simulink model "reinforcemen_model_realtest"  (R2023b)
settings: Solver=FixedStepAuto  StartTime=0.0  StopTime=inf  FixedStep=0.05  RelTol=1e-3
undefined symbols (not defined in the file or in its folder): saved_agent, Ts
libraries: arduinolib x10, rllib x5, dspstat3 x5, dxlSimLibrary x4, simulink x2
settings Model: SimulationMode=accelerator  ExtModeTrigDuration=2  VariantFading=off  Creator=MSI PC  LastModifiedBy=Yuk
settings OptimizationCC: EnhancedBackFolding=on  PassReuseOutputArgsAs=Individual arguments  ZeroExternalMemoryAtStartup=off  ZeroInternalMemoryAtStartup=off  MaxStackSize=64  OptimizeBlockOrder=speed  DifferentSizesBufferReuse=on  OptimizationCustomize=off  EfficientTunableParamExpr=on
settings DebuggingCC: MultiTaskRateTransMsg=warning  ParameterPrecisionLossMsg=none  ParameterTunabilityLossMsg=error  UnconnectedInputMsg=warning  UnconnectedOutputMsg=warning  UnconnectedLineMsg=warning
settings HardwareCC: ProdBitPerInt=16  ProdBitPerPointer=16  ProdBitPerSizeT=16  ProdBitPerPtrDiffT=16  ProdLargestAtomicFloat=None  ProdWordSize=8  ProdHWDeviceType=Atmel->AVR
settings ModelReferenceCC: EnableRefExpFcnMdlSchedulingChecks=on
settings SFSimCC: MATLABDynamicMemAlloc=off
settings RTWCC: Description=Embedded Coder  SystemTargetFile=ert.tlc  HardwareBoard=Arduino Uno  TemplateMakefile=ert_default_tmf  Toolchain=Arduino AVR  BuildConfiguration=Faster Runs  DLArmComputeVersion=19.05
settings CodeAppCC: ForceParamTrailComments=on  IgnoreCustomStorageClasses=off  OperatorAnnotations=on  SimulinkDataObjDesc=on  SFDataObjDesc=on  InsertBlockDesc=on
settings ERTTargetCC: SupportContinuousTime=on  SupportVariableSizeSignals=on  ExtModeTransport=3  ExtModeStaticAlloc=on  ExtModeAutomaticAllocSize=off  ExtModeStaticAllocSize=250  ExtModeMexFile=ext_xcp  ExtModeIntrfLevel=Level2 - Open

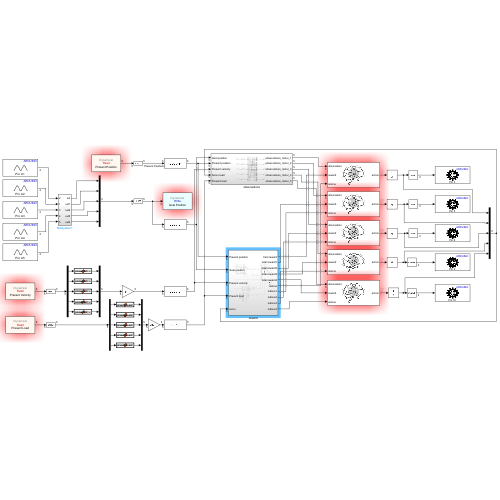
[thumbnail: Simulink's stored preview of the top-level diagram]
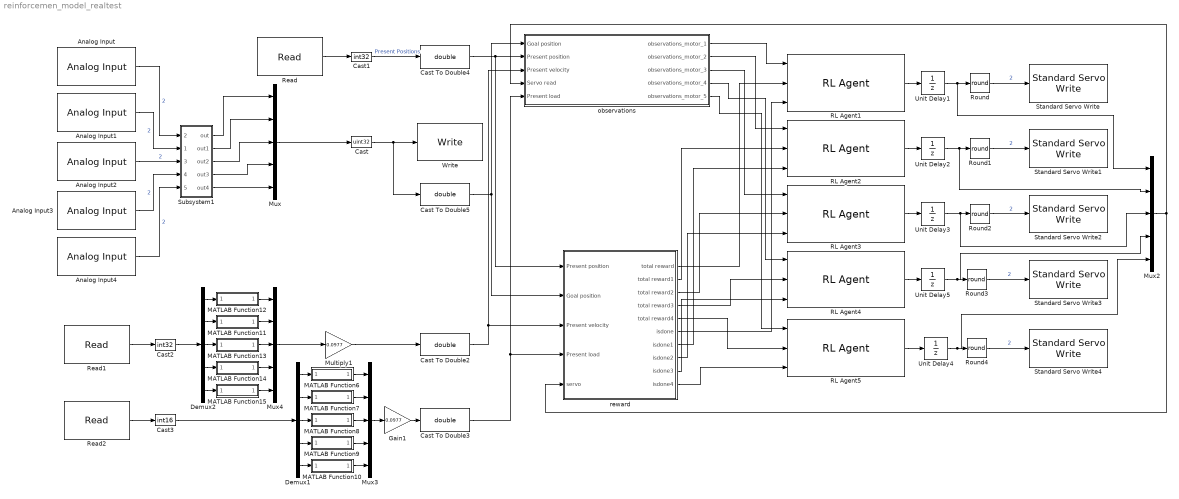
== system reinforcemen_model_realtest ==
  Analog Input : arduinolib/Analog Input  pinNumber=1  ReadResultsOnly=off  ConversionTriggerSource=Software  ExternalTriggerType=uint32( 0 )  OutputDataType=uint16  EnableConversionCompleteNotify=off  EnableOuputStatus=off  SampleTime=0.05  blockPlatform=arduino
  Analog Input1 : arduinolib/Analog Input  pinNumber=2  ReadResultsOnly=off  ConversionTriggerSource=Software  ExternalTriggerType=uint32( 0 )  OutputDataType=uint16  EnableConversionCompleteNotify=off  EnableOuputStatus=off  SampleTime=0.05  blockPlatform=arduino
  Analog Input2 : arduinolib/Analog Input  pinNumber=3  ReadResultsOnly=off  ConversionTriggerSource=Software  ExternalTriggerType=uint32( 0 )  OutputDataType=uint16  EnableConversionCompleteNotify=off  EnableOuputStatus=off  SampleTime=0.05  blockPlatform=arduino
  Analog Input3 : arduinolib/Analog Input  pinNumber=4  ReadResultsOnly=off  ConversionTriggerSource=Software  ExternalTriggerType=uint32( 0 )  OutputDataType=uint16  EnableConversionCompleteNotify=off  EnableOuputStatus=off  SampleTime=0.05  blockPlatform=arduino
  Analog Input4 : arduinolib/Analog Input  pinNumber=5  ReadResultsOnly=off  ConversionTriggerSource=Software  ExternalTriggerType=uint32( 0 )  OutputDataType=uint16  EnableConversionCompleteNotify=off  EnableOuputStatus=off  SampleTime=0.05  blockPlatform=arduino
  Cast : DataTypeConversion  OutMin=0  OutMax=2097150  OutDataTypeStr=uint32  SaturateOnIntegerOverflow=off  RndMeth=Floor
  Cast To Double{2..5} (4 alike) : DataTypeConversion  OutDataTypeStr=double  SaturateOnIntegerOverflow=off  RndMeth=Floor
  Cast1 : DataTypeConversion  OutDataTypeStr=int32  SaturateOnIntegerOverflow=off  RndMeth=Floor
  Cast2 : DataTypeConversion  OutDataTypeStr=int32  SaturateOnIntegerOverflow=off  RndMeth=Floor
  Cast3 : DataTypeConversion  OutDataTypeStr=int16  SaturateOnIntegerOverflow=off  RndMeth=Floor
  Demux1 : Demux  Outputs=5
  Demux2 : Demux  Outputs=5
  Gain1 : Gain  Gain=0.0977
  MATLAB Function10 : MATLAB Function  TreatAsAtomicUnit=on
  MATLAB Function11 : MATLAB Function  TreatAsAtomicUnit=on
  MATLAB Function12 : MATLAB Function  TreatAsAtomicUnit=on
  MATLAB Function13 : MATLAB Function  TreatAsAtomicUnit=on
  MATLAB Function14 : MATLAB Function  TreatAsAtomicUnit=on
  MATLAB Function15 : MATLAB Function  TreatAsAtomicUnit=on
  MATLAB Function6 : MATLAB Function  TreatAsAtomicUnit=on
  MATLAB Function7 : MATLAB Function  TreatAsAtomicUnit=on
  MATLAB Function8 : MATLAB Function  TreatAsAtomicUnit=on
  MATLAB Function9 : MATLAB Function  TreatAsAtomicUnit=on
  Multiply1 : Gain  Gain=0.0977  OutDataTypeStr=double
  Mux{,2..4} (4 alike) : Mux  Inputs=5
  RL Agent1 : rllib/RL Agent  Agent=saved_agent(1,1)  ExternalActionAsInput=off  ProvideLastAction=off  ProvideCumRwd=off  TreatAsDirectFeedthrough=on  UseStrictObservationDataTypes=off
  RL Agent2 : rllib/RL Agent  Agent=saved_agent(1,2)  ExternalActionAsInput=off  ProvideLastAction=off  ProvideCumRwd=off  TreatAsDirectFeedthrough=on  UseStrictObservationDataTypes=off
  RL Agent3 : rllib/RL Agent  Agent=saved_agent(1,3)  ExternalActionAsInput=off  ProvideLastAction=off  ProvideCumRwd=off  TreatAsDirectFeedthrough=on  UseStrictObservationDataTypes=off
  RL Agent4 : rllib/RL Agent  Agent=saved_agent(1,4)  ExternalActionAsInput=off  ProvideLastAction=off  ProvideCumRwd=off  TreatAsDirectFeedthrough=on  UseStrictObservationDataTypes=off
  RL Agent5 : rllib/RL Agent  Agent=saved_agent(1,5)  ExternalActionAsInput=off  ProvideLastAction=off  ProvideCumRwd=off  TreatAsDirectFeedthrough=on  UseStrictObservationDataTypes=off
  Read : dxlSimLibrary/Read  lib_name=lib_name  port_num=port_num  protocol_version=protocol_version  ids=motor_IDs  models=motor_models  select=Present Position  Ts=Ts
  Read1 : dxlSimLibrary/Read  lib_name=lib_name  port_num=port_num  protocol_version=protocol_version  ids=motor_IDs  models=motor_models  select=Present Velocity  Ts=Ts
  Read2 : dxlSimLibrary/Read  lib_name=lib_name  port_num=port_num  protocol_version=protocol_version  ids=motor_IDs  models=motor_models  select=Present Load  Ts=Ts
  Round{,1..4} (5 alike) : Rounding  Operator=round
  Standard Servo Write : arduinolib/Standard Servo Write  pinNumber=3  ServoIndex=0  blockPlatform=ARDUINO
  Standard Servo Write1 : arduinolib/Standard Servo Write  pinNumber=5  ServoIndex=1  blockPlatform=ARDUINO
  Standard Servo Write2 : arduinolib/Standard Servo Write  pinNumber=6  ServoIndex=2  blockPlatform=ARDUINO
  Standard Servo Write3 : arduinolib/Standard Servo Write  pinNumber=9  ServoIndex=3  blockPlatform=ARDUINO
  Standard Servo Write4 : arduinolib/Standard Servo Write  pinNumber=10  ServoIndex=4  blockPlatform=ARDUINO
  Subsystem1 : Subsystem
  Unit Delay1 : UnitDelay  SampleTime=-1  HasFrameUpgradeWarning=on
  Unit Delay{2..5} (4 alike) : UnitDelay  InitialCondition=180  SampleTime=-1  HasFrameUpgradeWarning=on
  Write : dxlSimLibrary/Write  lib_name=lib_name  port_num=port_num  protocol_version=protocol_version  ids=motor_IDs  models=motor_models  select=Goal Position  Ts=Ts
  observations : Subsystem
  reward : Subsystem
  wires:
  observations/5(observations_motor_5) -> RL Agent5/1
  Cast2/1 -> Demux2/1
  Cast3/1 -> Demux1/1
  Read1/1 -> Cast2/1
  Read2/1 -> Cast3/1
  Analog Input/1 -> Subsystem1/1(2)  "2"
  Analog Input1/1 -> Subsystem1/2(1)  "2"
  Analog Input4/1 -> Subsystem1/5(5)  "2"
  Analog Input2/1 -> Subsystem1/3(3)  "2"
  Analog Input3/1 -> Subsystem1/4(4)  "2"
  Demux2/1 -> MATLAB Function12/1(presentVel)
  Demux2/5 -> MATLAB Function15/1(presentVel)
  Demux2/4 -> MATLAB Function14/1(presentVel)
  Demux2/3 -> MATLAB Function13/1(presentVel)
  Demux2/2 -> MATLAB Function11/1(presentVel)
  Demux1/3 -> MATLAB Function8/1(presentLoad)
  Demux1/2 -> MATLAB Function7/1(presentLoad)
  Demux1/1 -> MATLAB Function6/1(presentLoad)
  Gain1/1 -> Cast To Double3/1
  Demux1/5 -> MATLAB Function10/1(presentLoad)
  Demux1/4 -> MATLAB Function9/1(presentLoad)
  Mux/1 -> Cast/1
  Subsystem1/5(out4) -> Mux/5
  Subsystem1/1(out) -> Mux/1
  Subsystem1/3(out2) -> Mux/3
  Subsystem1/2(out1) -> Mux/2
  Subsystem1/4(out3) -> Mux/4
  MATLAB Function14/1(convertedVel) -> Mux4/4
  MATLAB Function13/1(convertedVel) -> Mux4/3
  MATLAB Function11/1(convertedVel) -> Mux4/2
  MATLAB Function12/1(convertedVel) -> Mux4/1
  reward/6(isdone) -> RL Agent1/3
  Multiply1/1 -> Cast To Double2/1
  MATLAB Function15/1(convertedVel) -> Mux4/5
  MATLAB Function10/1(convertedLoad) -> Mux3/5
  MATLAB Function8/1(convertedLoad) -> Mux3/3
  MATLAB Function7/1(convertedLoad) -> Mux3/2
  MATLAB Function6/1(convertedLoad) -> Mux3/1
  RL Agent2/1 -> Unit Delay2/1
  MATLAB Function9/1(convertedLoad) -> Mux3/4
  Read/1 -> Cast1/1
  Mux4/1 -> Multiply1/1
  Mux3/1 -> Gain1/1
  reward/3(total reward2) -> RL Agent3/2
  Cast1/1 -> Cast To Double4/1  "Present Positions"
  reward/4(total reward3) -> RL Agent4/2
  Cast/1 -> Write/1, Cast To Double5/1
  Cast To Double5/1 -> reward/2(Goal position), observations/1(Goal position)
  reward/5(total reward4) -> RL Agent5/2
  Cast To Double4/1 -> reward/1(Present position), observations/2(Present position)
  Cast To Double2/1 -> reward/3(Present velocity), observations/3(Present velocity)
  RL Agent3/1 -> Unit Delay3/1
  observations/1(observations_motor_1) -> RL Agent1/1
  observations/2(observations_motor_2) -> RL Agent2/1
  observations/3(observations_motor_3) -> RL Agent3/1
  observations/4(observations_motor_4) -> RL Agent4/1
  reward/1(total reward) -> RL Agent1/2
  reward/2(total reward1) -> RL Agent2/2
  reward/7(isdone1) -> RL Agent2/3
  reward/8(isdone2) -> RL Agent3/3
  reward/9(isdone3) -> RL Agent4/3
  reward/10(isdone4) -> RL Agent5/3
  RL Agent4/1 -> Unit Delay5/1
  RL Agent5/1 -> Unit Delay4/1
  Round1/1 -> Standard Servo Write1/1  "2"
  RL Agent1/1 -> Unit Delay1/1
  Round2/1 -> Standard Servo Write2/1  "2"
  Round3/1 -> Standard Servo Write3/1  "2"
  Round4/1 -> Standard Servo Write4/1  "2"
  Round/1 -> Standard Servo Write/1  "2"
  Mux2/1 -> reward/5(servo), observations/4(Servo read)
  Unit Delay5/1 -> Mux2/4, Round3/1
  Unit Delay4/1 -> Mux2/5, Round4/1
  Unit Delay1/1 -> Round/1, Mux2/1
  Cast To Double3/1 -> reward/4(Present load), observations/5(Present load)
  Unit Delay3/1 -> Mux2/3, Round2/1
  Unit Delay2/1 -> Mux2/2, Round1/1

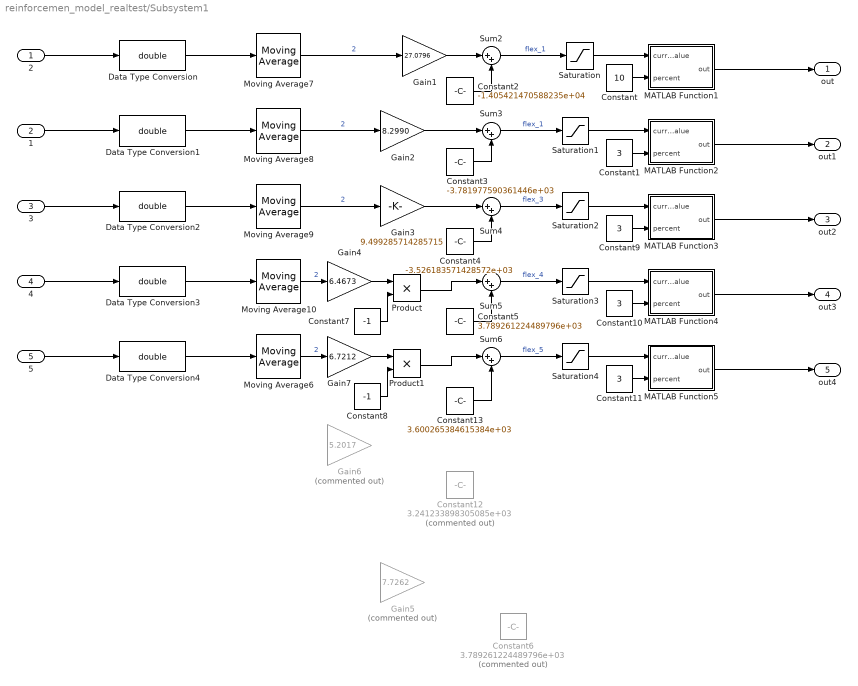
== system reinforcemen_model_realtest/Subsystem1 ==
  2 : Inport
  1 : Inport  Port=2
  3 : Inport  Port=3
  4 : Inport  Port=4
  5 : Inport  Port=5
  Constant : Constant  Value=10
  Constant{1,9..11} (4 alike) : Constant  Value=3
  Constant12 : Constant  Commented=on  Value=3.241233898305085e+03
  Constant13 : Constant  Value=3.600265384615384e+03
  Constant2 : Constant  Value=-1.405421470588235e+04
  Constant3 : Constant  Value=-3.781977590361446e+03
  Constant4 : Constant  Value=-3.526183571428572e+03
  Constant5 : Constant  Value=3.789261224489796e+03
  Constant6 : Constant  Commented=on  Value=3.789261224489796e+03
  Constant7 : Constant  Value=-1
  Constant8 : Constant  Value=-1
  Data Type Conversion{,1..4} (5 alike) : DataTypeConversion  OutDataTypeStr=double  SaturateOnIntegerOverflow=off  RndMeth=Floor
  Gain1 : Gain  Gain=27.0796
  Gain2 : Gain  Gain=8.2990
  Gain3 : Gain  Gain=9.499285714285715
  Gain4 : Gain  Gain=6.4673
  Gain5 : Gain  Commented=on  Gain=7.7262
  Gain6 : Gain  Commented=on  Gain=5.2017
  Gain7 : Gain  Gain=6.7212
  MATLAB Function1 : MATLAB Function  TreatAsAtomicUnit=on
  MATLAB Function2 : MATLAB Function  TreatAsAtomicUnit=on
  MATLAB Function3 : MATLAB Function  TreatAsAtomicUnit=on
  MATLAB Function4 : MATLAB Function  TreatAsAtomicUnit=on
  MATLAB Function5 : MATLAB Function  TreatAsAtomicUnit=on
  Moving Average{6..10} (5 alike) : dspstat3/Moving Average  Method=Sliding window  ForgettingFactorPort=off  SpecifyWindowLength=on  WindowLength=3  OverlapLength=2  AllowArbitraryInputLength=off  ForgettingFactor=0.9  SimulateUsing=Code generation
  Product : Product
  Product1 : Product
  Saturation : Saturate  UpperLimit=920.7  LowerLimit=0
  Saturation1 : Saturate  UpperLimit=716.1  LowerLimit=27.28
  Saturation2 : Saturate  UpperLimit=640  LowerLimit=17.05
  Saturation3 : Saturate  UpperLimit=988.9  LowerLimit=375.1
  Saturation4 : Saturate  UpperLimit=1005.9  LowerLimit=306.9
  Sum{2..6} (5 alike) : Sum  Inputs=|++
  out : Outport
  out1 : Outport  Port=2
  out2 : Outport  Port=3
  out3 : Outport  Port=4
  out4 : Outport  Port=5
  wires:
  3/1 -> Data Type Conversion2/1
  5/1 -> Data Type Conversion4/1
  MATLAB Function4/1(out) -> out3/1
  MATLAB Function1/1(out) -> out/1
  MATLAB Function2/1(out) -> out1/1
  1/1 -> Data Type Conversion1/1
  Constant5/1 -> Sum5/2
  Constant9/1 -> MATLAB Function3/2(percent)
  Constant/1 -> MATLAB Function1/2(percent)
  Constant10/1 -> MATLAB Function4/2(percent)
  Sum5/1 -> Saturation3/1  "flex_4"
  Saturation/1 -> MATLAB Function1/1(currentValue)
  4/1 -> Data Type Conversion3/1
  Constant4/1 -> Sum4/2
  Moving Average6/1 -> Gain7/1  "2"
  Gain2/1 -> Sum3/1
  Constant1/1 -> MATLAB Function2/2(percent)
  MATLAB Function5/1(out) -> out4/1
  Constant8/1 -> Product1/2
  Moving Average9/1 -> Gain3/1  "2"
  Constant3/1 -> Sum3/2
  Product1/1 -> Sum6/1
  Saturation4/1 -> MATLAB Function5/1(currentValue)
  MATLAB Function3/1(out) -> out2/1
  Moving Average7/1 -> Gain1/1  "2"
  Data Type Conversion2/1 -> Moving Average9/1
  Data Type Conversion/1 -> Moving Average7/1
  Data Type Conversion4/1 -> Moving Average6/1
  Gain1/1 -> Sum2/1
  Saturation3/1 -> MATLAB Function4/1(currentValue)
  Moving Average8/1 -> Gain2/1  "2"
  Gain4/1 -> Product/1
  Constant11/1 -> MATLAB Function5/2(percent)
  Sum4/1 -> Saturation2/1  "flex_3"
  Saturation2/1 -> MATLAB Function3/1(currentValue)
  Data Type Conversion1/1 -> Moving Average8/1
  Sum3/1 -> Saturation1/1  "flex_1"
  Sum2/1 -> Saturation/1  "flex_1"
  Saturation1/1 -> MATLAB Function2/1(currentValue)
  Constant7/1 -> Product/2
  2/1 -> Data Type Conversion/1
  Constant2/1 -> Sum2/2
  Gain3/1 -> Sum4/1
  Sum6/1 -> Saturation4/1  "flex_5"
  Gain7/1 -> Product1/1
  Data Type Conversion3/1 -> Moving Average10/1
  Moving Average10/1 -> Gain4/1  "2"
  Constant13/1 -> Sum6/2
  Product/1 -> Sum5/1

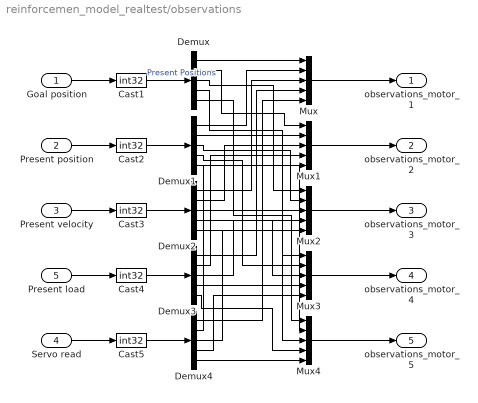
== system reinforcemen_model_realtest/observations ==
  Goal position : Inport
  Present position : Inport  Port=2
  Present velocity : Inport  Port=3
  Servo read : Inport  Port=4
  Present load : Inport  Port=5
  Cast{1..5} (5 alike) : DataTypeConversion  OutDataTypeStr=int32  SaturateOnIntegerOverflow=off  RndMeth=Floor
  Demux{,1..4} (5 alike) : Demux  Outputs=5
  Mux{,1..4} (5 alike) : Mux  Inputs=5
  observations_motor_1 : Outport
  observations_motor_2 : Outport  Port=2
  observations_motor_3 : Outport  Port=3
  observations_motor_4 : Outport  Port=4
  observations_motor_5 : Outport  Port=5
  wires:
  Goal position/1 -> Cast1/1
  Present position/1 -> Cast2/1
  Present velocity/1 -> Cast3/1
  Present load/1 -> Cast4/1
  Servo read/1 -> Cast5/1
  Demux/1 -> Mux/1
  Demux1/1 -> Mux/2
  Demux2/1 -> Mux/3
  Demux3/1 -> Mux/4
  Demux4/1 -> Mux/5
  Demux/2 -> Mux1/1
  Demux1/2 -> Mux1/2
  Demux2/2 -> Mux1/3
  Demux3/2 -> Mux1/4
  Demux4/2 -> Mux1/5
  Demux/3 -> Mux2/1
  Demux1/3 -> Mux2/2
  Demux2/3 -> Mux2/3
  Demux3/3 -> Mux2/4
  Demux4/3 -> Mux2/5
  Demux/4 -> Mux3/1
  Demux1/4 -> Mux3/2
  Demux2/4 -> Mux3/3
  Demux3/4 -> Mux3/4
  Demux4/4 -> Mux3/5
  Demux/5 -> Mux4/1
  Demux1/5 -> Mux4/2
  Demux2/5 -> Mux4/3
  Demux3/5 -> Mux4/4
  Demux4/5 -> Mux4/5
  Mux/1 -> observations_motor_1/1
  Mux1/1 -> observations_motor_2/1
  Mux2/1 -> observations_motor_3/1
  Mux3/1 -> observations_motor_4/1
  Mux4/1 -> observations_motor_5/1
  Cast2/1 -> Demux1/1
  Cast3/1 -> Demux2/1
  Cast4/1 -> Demux3/1
  Cast5/1 -> Demux4/1
  Cast1/1 -> Demux/1  "Present Positions"

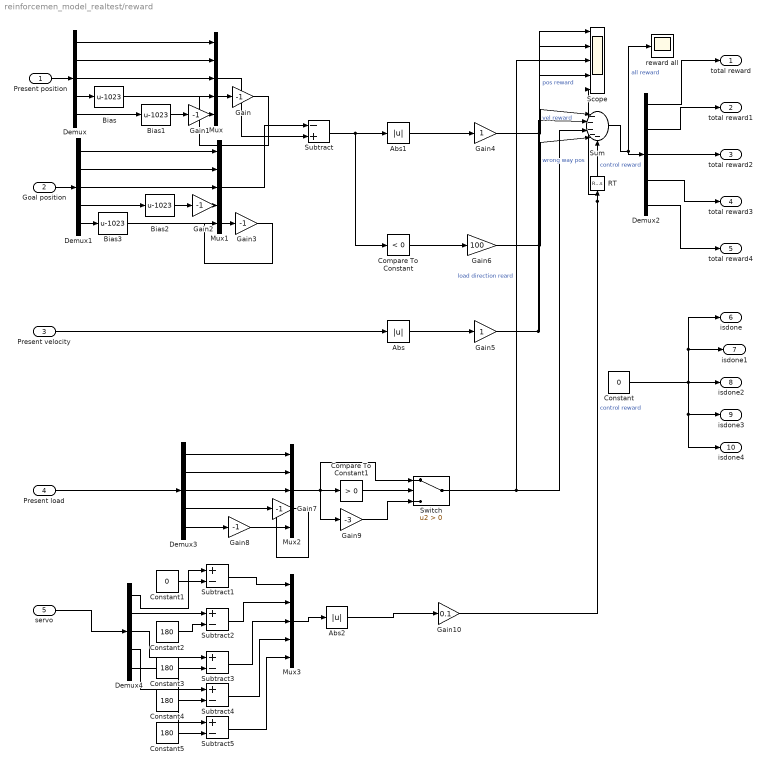
== system reinforcemen_model_realtest/reward ==
  Present position : Inport
  Goal position : Inport  Port=2
  Present velocity : Inport  Port=3
  Present load : Inport  Port=4
  servo : Inport  Port=5
  Abs : Abs  SaturateOnIntegerOverflow=off
  Abs1 : Abs  SaturateOnIntegerOverflow=off
  Abs2 : Abs  SaturateOnIntegerOverflow=off
  Bias{,1..3} (4 alike) : Bias  Bias=-1023  SaturateOnIntegerOverflow=off
  Compare To Constant : simulink/Logic and Bit Operations/Compare To Constant  relop=<  const=0  OutDataTypeStr=boolean
  Compare To Constant1 : simulink/Logic and Bit Operations/Compare To Constant  relop=>  const=0  OutDataTypeStr=boolean
  Constant : Constant  Value=0
  Constant1 : Constant  Value=0
  Constant{2..5} (4 alike) : Constant  Value=180
  Demux{,1..4} (5 alike) : Demux  Outputs=5
  Gain{,1..3,7..8} (6 alike) : Gain  Gain=-1
  Gain10 : Gain  Gain=0.1
  Gain4 : Gain
  Gain5 : Gain
  Gain6 : Gain  Gain=100
  Gain9 : Gain  Gain=-3
  Mux{,1..3} (4 alike) : Mux  Inputs=5
  RT : RateTransition  OutPortSampleTime=0.05
  Scope : Scope  NumInputPorts=5
  Subtract : Sum  Inputs=-+
  Subtract{1..5} (5 alike) : Sum  Inputs=+-
  Sum : Sum  Inputs=|-----
  Switch : Switch  Criteria=u2 > Threshold  SaturateOnIntegerOverflow=off  InputSameDT=off
  reward all : Scope
  total reward : Outport
  total reward1 : Outport  Port=2
  total reward2 : Outport  Port=3
  total reward3 : Outport  Port=4
  total reward4 : Outport  Port=5
  isdone : Outport  Port=6
  isdone1 : Outport  Port=7
  isdone2 : Outport  Port=8
  isdone3 : Outport  Port=9
  isdone4 : Outport  Port=10
  wires:
  Present velocity/1 -> Abs/1
  Present position/1 -> Demux/1
  Demux/5 -> Bias1/1
  Demux/4 -> Bias/1
  Demux/3 -> Mux/3
  Demux/2 -> Mux/2
  Demux/1 -> Mux/1
  Bias/1 -> Gain/1
  Bias1/1 -> Gain1/1
  Gain/1 -> Mux/4
  Gain1/1 -> Mux/5
  Gain3/1 -> Mux1/5
  Gain2/1 -> Mux1/4
  Bias3/1 -> Gain3/1
  Bias2/1 -> Gain2/1
  Demux1/1 -> Mux1/1
  Demux1/2 -> Mux1/2
  Demux1/3 -> Mux1/3
  Demux1/4 -> Bias2/1
  Demux1/5 -> Bias3/1
  Goal position/1 -> Demux1/1
  Mux1/1 -> Subtract/1
  Mux/1 -> Subtract/2
  Subtract/1 -> Compare To Constant/1, Abs1/1
  Abs1/1 -> Gain4/1
  Gain4/1 -> Scope/1, Sum/1  "pos reward"
  Abs/1 -> Gain5/1
  Gain5/1 -> Scope/2, Sum/2  "vel reward"
  Present load/1 -> Demux3/1
  Compare To Constant/1 -> Gain6/1
  Gain6/1 -> Scope/4, Sum/4  "wrong way pos"
  Constant/1 -> isdone4/1, isdone3/1, isdone/1, isdone1/1, isdone2/1
  Sum/1 -> Demux2/1, reward all/1  "all reward"
  Demux2/3 -> total reward2/1
  Demux2/2 -> total reward1/1
  Demux2/1 -> total reward/1
  Demux2/4 -> total reward3/1
  Demux2/5 -> total reward4/1
  Demux3/4 -> Gain7/1
  Demux3/1 -> Mux2/1
  Demux3/3 -> Mux2/3
  Demux3/5 -> Gain8/1
  Gain7/1 -> Mux2/4
  Demux3/2 -> Mux2/2
  Gain8/1 -> Mux2/5
  Mux2/1 -> Gain9/1, Switch/1, Compare To Constant1/1
  Compare To Constant1/1 -> Switch/2
  Gain9/1 -> Switch/3
  Switch/1 -> Scope/3, Sum/3  "load direction reard"
  servo/1 -> Demux4/1
  Abs2/1 -> Gain10/1
  Demux4/5 -> Subtract5/1
  Demux4/2 -> Subtract2/1
  Demux4/4 -> Subtract4/1
  Demux4/1 -> Subtract1/1
  Demux4/3 -> Subtract3/1
  Constant1/1 -> Subtract1/2
  Constant2/1 -> Subtract2/2
  Constant3/1 -> Subtract3/2
  Constant4/1 -> Subtract4/2
  Constant5/1 -> Subtract5/2
  Subtract3/1 -> Mux3/3
  Subtract2/1 -> Mux3/2
  Subtract1/1 -> Mux3/1
  Subtract4/1 -> Mux3/4
  Subtract5/1 -> Mux3/5
  Mux3/1 -> Abs2/1
  Gain10/1 -> Scope/5, RT/1  "control reward"
  RT/1 -> Sum/5  "control reward"

== matlab function reinforcemen_model_realtest/MATLAB Function14 ==
  data: presentVel input; convertedVel output
function convertedVel = convertVel(presentVel)
% Convert Dynamixel present load data from 0-2047 to -1023 to 1023
% 0-1023 remains as is, 1024-2047 is mapped to 0 to -1023

if presentVel >= 1024
    convertedVel = -(presentVel - 1024);
else
    convertedVel = presentVel;
end
end

== matlab function reinforcemen_model_realtest/MATLAB Function15 ==
  data: presentVel input; convertedVel output
function convertedVel = convertVel(presentVel)
% Convert Dynamixel present load data from 0-2047 to -1023 to 1023
% 0-1023 remains as is, 1024-2047 is mapped to 0 to -1023

if presentVel >= 1024
    convertedVel = -(presentVel - 1024);
else
    convertedVel = presentVel;
end
end

== matlab function reinforcemen_model_realtest/Subsystem1/MATLAB Function1 ==
  data: currentValue input; out output; percent input
function out = customDeadZone(currentValue,percent)
    % 지속적인 상태 유지를 위한 영구 변수 선언
    persistent lastValue
    if isempty(lastValue)
        lastValue = currentValue; % 최초 실행 시 초기값 설정
    end
    
    % 변화 임계값 설정
    threshold = (percent*682)/100;
    
    % 현재 값과 이전 값의 차이가 임계값보다 크면 업데이트
    if abs(currentValue - lastValue) > threshold
        lastValue = currentValue; % 값 업데이트
    end
    
    % 출력
    out = lastValue;
end

== matlab function reinforcemen_model_realtest/Subsystem1/MATLAB Function3 ==
  data: currentValue input; out output; percent input
function out = customDeadZone(currentValue,percent)
    % 지속적인 상태 유지를 위한 영구 변수 선언
    persistent lastValue
    if isempty(lastValue)
        lastValue = currentValue; % 최초 실행 시 초기값 설정
    end
    
    % 변화 임계값 설정
    threshold = (percent*682)/100;
    
    % 현재 값과 이전 값의 차이가 임계값보다 크면 업데이트
    if abs(currentValue - lastValue) > threshold
        lastValue = currentValue; % 값 업데이트
    end
    
    % 출력
    out = lastValue;
end

== matlab function reinforcemen_model_realtest/Subsystem1/MATLAB Function4 ==
  data: currentValue input; out output; percent input
function out = customDeadZone(currentValue,percent)
    % 지속적인 상태 유지를 위한 영구 변수 선언
    persistent lastValue
    if isempty(lastValue)
        lastValue = currentValue; % 최초 실행 시 초기값 설정
    end
    
    % 변화 임계값 설정
    threshold = (percent*682)/100;
    
    % 현재 값과 이전 값의 차이가 임계값보다 크면 업데이트
    if abs(currentValue - lastValue) > threshold
        lastValue = currentValue; % 값 업데이트
    end
    
    % 출력
    out = lastValue;
end

== matlab function reinforcemen_model_realtest/Subsystem1/MATLAB Function5 ==
  data: currentValue input; out output; percent input
function out = customDeadZone(currentValue,percent)
    % 지속적인 상태 유지를 위한 영구 변수 선언
    persistent lastValue
    if isempty(lastValue)
        lastValue = currentValue; % 최초 실행 시 초기값 설정
    end
    
    % 변화 임계값 설정
    threshold = (percent*682)/100;
    
    % 현재 값과 이전 값의 차이가 임계값보다 크면 업데이트
    if abs(currentValue - lastValue) > threshold
        lastValue = currentValue; % 값 업데이트
    end
    
    % 출력
    out = lastValue;
end

== matlab function reinforcemen_model_realtest/MATLAB Function6 ==
  data: presentLoad input; convertedLoad output
function convertedLoad = convertLoad(presentLoad)
% Convert Dynamixel present load data from 0-2047 to -1023 to 1023
% 0-1023 remains as is, 1024-2047 is mapped to 0 to -1023

if presentLoad >= 1024
    convertedLoad = -(presentLoad - 1024);
else
    convertedLoad = presentLoad;
end
end

== matlab function reinforcemen_model_realtest/MATLAB Function7 ==
  data: presentLoad input; convertedLoad output
function convertedLoad = convertLoad(presentLoad)
% Convert Dynamixel present load data from 0-2047 to -1023 to 1023
% 0-1023 remains as is, 1024-2047 is mapped to 0 to -1023

if presentLoad >= 1024
    convertedLoad = -(presentLoad - 1024);
else
    convertedLoad = presentLoad;
end
end

== matlab function reinforcemen_model_realtest/MATLAB Function8 ==
  data: presentLoad input; convertedLoad output
function convertedLoad = convertLoad(presentLoad)
% Convert Dynamixel present load data from 0-2047 to -1023 to 1023
% 0-1023 remains as is, 1024-2047 is mapped to 0 to -1023

if presentLoad >= 1024
    convertedLoad = -(presentLoad - 1024);
else
    convertedLoad = presentLoad;
end
end

== matlab function reinforcemen_model_realtest/MATLAB Function9 ==
  data: presentLoad input; convertedLoad output
function convertedLoad = convertLoad(presentLoad)
% Convert Dynamixel present load data from 0-2047 to -1023 to 1023
% 0-1023 remains as is, 1024-2047 is mapped to 0 to -1023

if presentLoad >= 1024
    convertedLoad = -(presentLoad - 1024);
else
    convertedLoad = presentLoad;
end
end

== matlab function reinforcemen_model_realtest/MATLAB Function10 ==
  data: presentLoad input; convertedLoad output
function convertedLoad = convertLoad(presentLoad)
% Convert Dynamixel present load data from 0-2047 to -1023 to 1023
% 0-1023 remains as is, 1024-2047 is mapped to 0 to -1023

if presentLoad >= 1024
    convertedLoad = -(presentLoad - 1024);
else
    convertedLoad = presentLoad;
end
end

== matlab function reinforcemen_model_realtest/Subsystem1/MATLAB Function2 ==
  data: currentValue input; out output; percent input
function out = customDeadZone(currentValue,percent)
    % 지속적인 상태 유지를 위한 영구 변수 선언
    persistent lastValue
    if isempty(lastValue)
        lastValue = currentValue; % 최초 실행 시 초기값 설정
    end
    
    % 변화 임계값 설정
    threshold = (percent*682)/100;
    
    % 현재 값과 이전 값의 차이가 임계값보다 크면 업데이트
    if abs(currentValue - lastValue) > threshold
        lastValue = currentValue; % 값 업데이트
    end
    
    % 출력
    out = lastValue;
end

== matlab function reinforcemen_model_realtest/MATLAB Function11 ==
  data: presentVel input; convertedVel output
function convertedVel = convertVel(presentVel)
% Convert Dynamixel present load data from 0-2047 to -1023 to 1023
% 0-1023 remains as is, 1024-2047 is mapped to 0 to -1023

if presentVel >= 1024
    convertedVel = -(presentVel - 1024);
else
    convertedVel = presentVel;
end
end

== matlab function reinforcemen_model_realtest/MATLAB Function12 ==
  data: presentVel input; convertedVel output
function convertedVel = convertVel(presentVel)
% Convert Dynamixel present load data from 0-2047 to -1023 to 1023
% 0-1023 remains as is, 1024-2047 is mapped to 0 to -1023

if presentVel >= 1024
    convertedVel = -(presentVel - 1024);
else
    convertedVel = presentVel;
end
end

== matlab function reinforcemen_model_realtest/MATLAB Function13 ==
  data: presentVel input; convertedVel output
function convertedVel = convertVel(presentVel)
% Convert Dynamixel present load data from 0-2047 to -1023 to 1023
% 0-1023 remains as is, 1024-2047 is mapped to 0 to -1023

if presentVel >= 1024
    convertedVel = -(presentVel - 1024);
else
    convertedVel = presentVel;
end
end
